simulink model "VIRTUAL_self_driving_stack_autoLocalize_v2"  (R2026a)
settings: Solver=ode1  StopTime=inf  FixedStep=1/500  EnableMultiTasking=on
values from neighbouring files (symbols this model uses):
  path_x4 = [-0.614 -0.604 -0.594 -0.584 -0.574 -0.564 -0.554 -0.544 -0.534 -0.524 -0.514 -0.504 ... (1761 elements, 1761x1)]    [SDCS_Paths_7.mat]
  path_y4 = [-1.0887 -1.0887 -1.0887 -1.0887 -1.0887 -1.0887 -1.0887 -1.0887 -1.0887 -1.0887 -1.0887 -1.0887 ... (1761 elements, 1761x1)]    [SDCS_Paths_7.mat]
undefined symbols (not defined in the file or in its folder): AAAF5050, CSI_Sample_Time, DiscIntNeverNeededParam, gcbh, height, HIL, ImageDisplay_Sample_Time, Initialization_Time, JPEG, K12, left, LiDAR_Sample_Time, MC, qc_get_step_size, RealSense_Sample_Time, top, video_display_show, width
libraries: quarc_library x67, simulink x5, visionconversions x1, visiontransforms x1, sl_discontinuities x1
(part 2 of 3)

== system VIRTUAL_self_driving_stack_autoLocalize_v2/readQCarDAC ==
  HIL Initialize : quarc_library/Data Acquisition/Generic/Configuration/HIL Initialize  object_name=HIL-2  board_type=qcar2  board_number=0@tcpip://localhost:18960  board_options=gyro_fs=250;gyro_rate=500;gyro_bw=125;gyro_ord=3;accel_fs=4;accel_rate=500;accel_bw=250;accel_ord=3;temp_bw=4000;enc0_dir=0;enc1_dir=0;enc2_dir=0;steer_bias=0.05;  exclusive=off  active=on  hardware_clocks=[]  clock_modes=[]  initial_clock_frequencies=[]  set_clock_params_at_start=off  set_clock_params_at_switch_in=off  set_clock_frequencies_at_start=off  set_clock_frequencies_at_switch_in=off  analog_input_channels=[0:4]  analog_input_configurations=[]  analog_input_maximums=[3.3]  analog_input_minimums=[0]  set_analog_input_params_at_start=off  set_analog_input_params_at_switch_in=off  analog_output_channels=[]  analog_output_maximums=[]  analog_output_minimums=[]  initial_analog_outputs=[]  final_analog_outputs=[]  watchdog_analog_outputs=[]  set_analog_output_params_at_start=off  set_analog_output_params_at_switch_in=off  set_analog_outputs_at_start=off  set_analog_outputs_at_switch_in=off  set_analog_outputs_at_terminate=off  set_analog_outputs_at_switch_out=off  set_analog_outputs_on_watchdog=off  digital_input_channels=[0:14]  digital_output_channels=[11:26]  digital_output_configuration=[]  initial_digital_outputs=[0]  final_digital_outputs=[0]  watchdog_digital_outputs=[0]  set_digital_output_params_at_start=off  set_digital_output_params_at_switch_in=off  set_digital_outputs_at_start=on  set_digital_outputs_at_switch_in=off  set_digital_outputs_at_terminate=on  set_digital_outputs_at_switch_out=off  set_digital_outputs_on_watchdog=off  encoder_channels=[0:2]  quadrature=[4]  encoder_filter_frequency=100e6/1  initial_encoder_counts=[0]  set_encoder_params_at_start=on  set_encoder_params_at_switch_in=off  set_encoder_counts_at_start=on  set_encoder_counts_at_switch_in=off  pwm_channels=[0:1]  pwm_modes=[0]  pwm_frequency=180e6/4096  pwm_configuration=[0]  pwm_alignment=[0]  pwm_polarity=[1]  pwm_leading_deadband=[]  pwm_trailing_deadband=[]  initial_pwm_outputs=[0]  final_pwm_outputs=[0]  watchdog_pwm_outputs=[0]  set_pwm_params_at_start=on  set_pwm_params_at_switch_in=off  set_pwm_outputs_at_start=on  set_pwm_outputs_at_switch_in=off  set_pwm_outputs_at_terminate=on  set_pwm_outputs_at_switch_out=off  set_pwm_outputs_on_watchdog=off  other_output_channels=[1000 11000]  initial_other_outputs=[0]  final_other_outputs=[0]  watchdog_other_outputs=[0]  set_other_outputs_at_start=on  set_other_outputs_at_switch_in=off  set_other_outputs_at_terminate=on  set_other_outputs_at_switch_out=off  set_other_outputs_on_watchdog=off
  HIL Read Timebase : quarc_library/Data Acquisition/Generic/Timebases/HIL Read Timebase  object_name=HIL-2  clock=0  analog_channels=[4 2]  encoder_channels=[0]  digital_channels=[]  other_channels=[3000:3002 4000:4002 14000]  active=on  vector_output=off  port_labels=channel numbers  data_type_mode=Inherit via back propagation  encoder_data_type=double  digital_data_type=boolean  overflow_mode=Synchronize (for simulated cards only)  samples_in_buffer=max(ceil(1/qc_get_step_size), 1)
  Mux1 : Mux  Inputs=3
  Mux2 : Mux  Inputs=3
  Unwrap 2^24 : quarc_library/Discontinuities/Inverse Modulus  modulus=16777215  output_derivative=off  output_revolutions=off  max_x=Inf  min_x=-Inf
  counts to meters : Subsystem
  counts/s to m/s : Subsystem
  powerConsumptionMonitor : Subsystem
  Speed (m/s) : Outport  VectorParamsAs1DForOutWhenUnconnected=off
  accelerometer (m/s^2) : Outport  Port=2  VectorParamsAs1DForOutWhenUnconnected=off
  gyroscope (rad/s) : Outport  Port=3  VectorParamsAs1DForOutWhenUnconnected=off
  odometer (m) : Outport  Port=4  VectorParamsAs1DForOutWhenUnconnected=off
  batteryVoltage (V) : Outport  Port=5
  motorCurrent (A) : Outport  Port=6
  batteryLevel (%) : Outport  Port=7
  motorPower (W) : Outport  Port=8
  wires:
  HIL Read Timebase/3 -> Unwrap 2^24/1  "encoder counts"
  HIL Read Timebase/1 -> powerConsumptionMonitor/1(motorCurrent (A) [1]), motorCurrent (A)/1  "motor current"
  HIL Read Timebase/2 -> batteryVoltage (V)/1, powerConsumptionMonitor/2(batteryVoltage (V) [1])  "battery voltage"
  HIL Read Timebase/10 -> counts/s to m/s/1(motorSpeed (counts/s))
  Unwrap 2^24/1 -> counts to meters/1(motorSpeed (counts/s))
  counts to meters/1(longitudinalCarSpeed (m/s)) -> odometer (m)/1
  counts/s to m/s/1(longitudinalCarSpeed (m/s)) -> Speed (m/s)/1
  powerConsumptionMonitor/1(motorPowerConsumption (W) [1]) -> motorPower (W)/1
  powerConsumptionMonitor/2(batteryLevel (%) [1]) -> batteryLevel (%)/1
  HIL Read Timebase/4 -> Mux1/1  "x"
  HIL Read Timebase/5 -> Mux1/2  "y"
  HIL Read Timebase/6 -> Mux1/3  "z"
  Mux1/1 -> gyroscope (rad/s)/1
  HIL Read Timebase/7 -> Mux2/1  "x"
  HIL Read Timebase/8 -> Mux2/2  "y"
  HIL Read Timebase/9 -> Mux2/3  "z"
  Mux2/1 -> accelerometer (m/s^2)/1

== system VIRTUAL_self_driving_stack_autoLocalize_v2/realsenseCapture ==
  Terminator{,1..4} (5 alike) : Terminator
  Video3D Initialize : quarc_library/Multimedia/Video3D Initialize  object_name=RealSense  source=Device  identifier=0@tcpip://localhost:18965  file=sample.bag  sample_time=RealSense_Sample_Time  active=on
  realsenseDepthCapture : quarc_library/Multimedia/Video3D Capture  object_name=RealSense  stream_type=Depth  stream_index=0  resolution=640 x 480  width=640  height=480  output_format=Distance in meters (HxW)  data_type=single  sample_time=RealSense_Sample_Time  camera_intrinsics=off  depth_scale=off  brightness_override=Do not override  brightness=50.0  contrast_override=Do not override  contrast=50.0  hue_override=Do not override  hue=50.0  saturation_override=Do not override  saturation=50.0  sharpness_override=Do not override  sharpness=50.0  gamma_override=Do not override  gamma=50.0  gain_override=Do not override  gain=50.0  backlightcompensation_override=Do not override  backlightcompensation=50.0  whitebalance_override=Automatic white balance  whitebalance=50.0  exposure_override=Automatic exposure  exposure=30.0  emitter=Enable laser emitter  preset=Do not set camera presets
  realsenseRGBCapture : quarc_library/Multimedia/Video3D Capture  object_name=RealSense  stream_type=RGB  stream_index=0  resolution=640 x 480  width=640  height=480  output_format=MATLAB RGB (HxWx3)  data_type=uint8  sample_time=RealSense_Sample_Time*1  camera_intrinsics=off  depth_scale=off  brightness_override=Do not override  brightness=50.0  contrast_override=Do not override  contrast=50.0  hue_override=Do not override  hue=50.0  saturation_override=Do not override  saturation=50.0  sharpness_override=Do not override  sharpness=50.0  gamma_override=Do not override  gamma=50.0  gain_override=Do not override  gain=50.0  backlightcompensation_override=Do not override  backlightcompensation=50.0  whitebalance_override=Automatic white balance  whitebalance=50.0  exposure_override=Automatic exposure  exposure=30.0  emitter=Enable laser emitter  preset=Do not set camera presets
  realsenseDepthImage [480 x 640] (single) : Outport
  newDepthImage [1] (bool) : Outport  Port=2
  "realsenseRGBImage [480 x 640] (uint8) " : Outport  Port=3
  newRGBImage [1] (bool) : Outport  Port=4
  wires:
  realsenseDepthCapture/4 -> newDepthImage [1] (bool)/1
  realsenseDepthCapture/2 -> Terminator4/1
  realsenseDepthCapture/3 -> Terminator3/1
  Video3D Initialize/1 -> Terminator/1
  realsenseRGBCapture/2 -> Terminator1/1
  realsenseRGBCapture/3 -> Terminator2/1
  realsenseRGBCapture/4 -> newRGBImage [1] (bool)/1
  realsenseRGBCapture/1 -> "realsenseRGBImage [480 x 640] (uint8) "/1
  realsenseDepthCapture/1 -> realsenseDepthImage [480 x 640] (single)/1

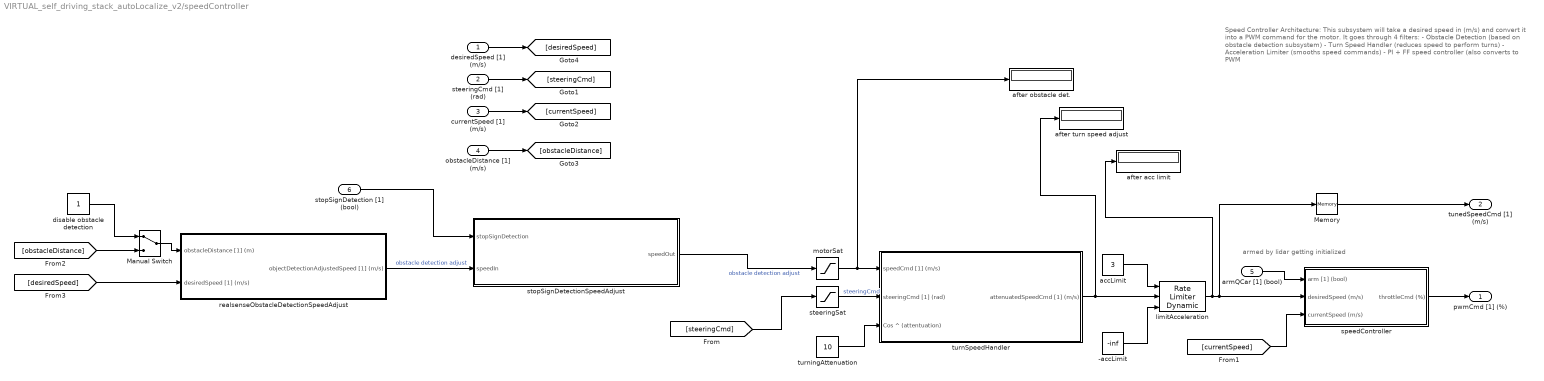
== system VIRTUAL_self_driving_stack_autoLocalize_v2/speedController ==
  note: Speed Controller Architecture:
      |
      | This subsystem will take a desired speed in (m/s) and convert it into a PWM command for the motor.
      |
      | It goes through 4 filters:
      | - Obstacle Detection (based on obstacle detection subsystem)
      | - Turn Speed Handler (reduces speed to perform turns)
      | - Acceleration Limiter (smooths speed commands)
      | - PI + FF speed controller (also converts to PWM
  note: armed by lidar getting initialized
  desiredSpeed [1] (m/s) : Inport
  steeringCmd [1] (rad) : Inport  Port=2
  currentSpeed [1] (m/s) : Inport  Port=3
  obstacleDistance [1] (m/s) : Inport  Port=4
  armQCar [1] (bool) : Inport  Port=5
  stopSignDetection [1] (bool) : Inport  Port=6
  -accLimit : Constant  Value=-inf
  Manual Switch : ManualSwitch
  Memory : Memory
  accLimit : Constant  Value=3
  after acc limit : Display
  after obstacle det. : Display
  after turn speed adjust : Display
  disable obstacle detection : Constant
  limitAcceleration : sl_discontinuities/Rate Limiter Dynamic
  motorSat : Saturate  UpperLimit=3  LowerLimit=-3
  realsenseObstacleDetectionSpeedAdjust : Subsystem
  speedController : Subsystem
  steeringSat : Saturate  UpperLimit=0.6  LowerLimit=-0.6
  stopSignDetectionSpeedAdjust : Subsystem
  turnSpeedHandler : Subsystem
  turningAttenuation : Constant  Value=10
  pwmCmd [1] (%) : Outport
  tunedSpeedCmd [1] (m/s) : Outport  Port=2
  wires:
  steeringSat/1 -> turnSpeedHandler/2(steeringCmd [1] (rad))  "steeringCmd"
  speedController/1(throttleCmd (%)) -> pwmCmd [1] (%)/1
  armQCar [1] (bool)/1 -> speedController/1(arm [1] (bool))
  turningAttenuation/1 -> turnSpeedHandler/3(Cos ^ (attentuation))
  motorSat/1 -> after obstacle det./1, turnSpeedHandler/1(speedCmd [1] (m/s))
  turnSpeedHandler/1(attenuatedSpeedCmd [1] (m/s)) -> after turn speed adjust/1, limitAcceleration/2
  accLimit/1 -> limitAcceleration/1
  limitAcceleration/1 -> after acc limit/1, Memory/1, speedController/2(desiredSpeed (m/s))
  -accLimit/1 -> limitAcceleration/3
  Memory/1 -> tunedSpeedCmd [1] (m/s)/1
  steeringCmd [1] (rad)/1 -> [steeringCmd]
  currentSpeed [1] (m/s)/1 -> [currentSpeed]
  [steeringCmd] -> steeringSat/1
  obstacleDistance [1] (m/s)/1 -> [obstacleDistance]
  [currentSpeed] -> speedController/3(currentSpeed (m/s))
  desiredSpeed [1] (m/s)/1 -> [desiredSpeed]
  [desiredSpeed] -> realsenseObstacleDetectionSpeedAdjust/2(desiredSpeed [1] (m/s))
  [obstacleDistance] -> Manual Switch/2
  disable obstacle detection/1 -> Manual Switch/1
  Manual Switch/1 -> realsenseObstacleDetectionSpeedAdjust/1(obstacleDistance [1] (m))
  stopSignDetection [1] (bool)/1 -> stopSignDetectionSpeedAdjust/1(stopSignDetection)
  realsenseObstacleDetectionSpeedAdjust/1(objectDetectionAdjustedSpeed [1] (m/s)) -> stopSignDetectionSpeedAdjust/2(speedIn)  "obstacle detection adjust"
  stopSignDetectionSpeedAdjust/1(speedOut) -> motorSat/1  "obstacle detection adjust"

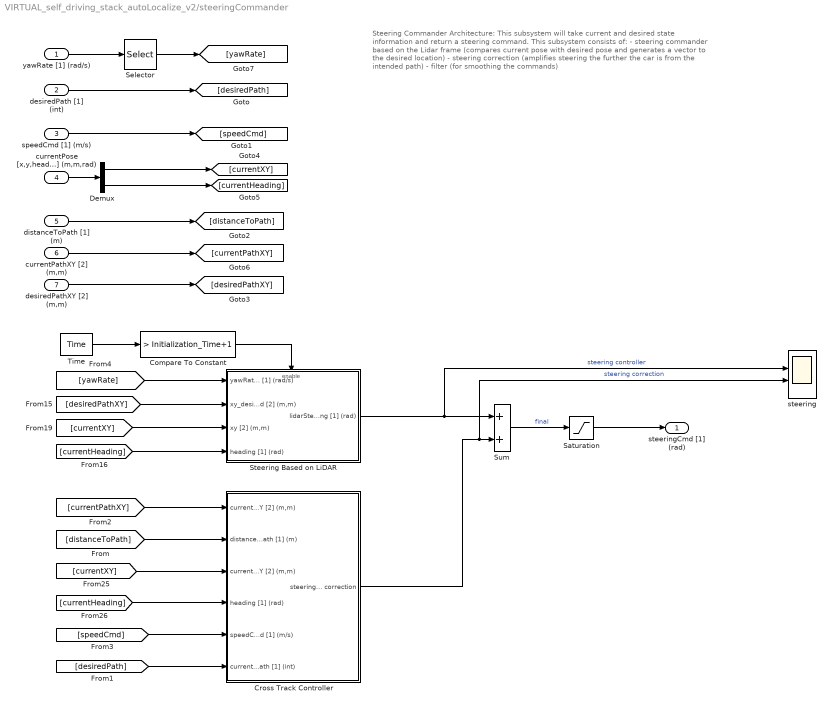
== system VIRTUAL_self_driving_stack_autoLocalize_v2/steeringCommander ==
  note: Steering Commander Architecture:
      |
      | This subsystem will take current and desired state information and return a steering command.
      |
      | This subsystem consists of:
      |
      | - steering commander based on the Lidar frame (compares current pose with desired pose and generates a vector to the desired location)
      | - steering correction (amplifies steering the further the car is from the intended path)
      | - filter (for smoothing the commands)
  yawRate [1] (rad/s) : Inport
  desiredPath [1] (int) : Inport  Port=2
  speedCmd [1] (m/s) : Inport  Port=3
  currentPose [x,y,heading] (m,m,rad) : Inport  Port=4
  distanceToPath [1] (m) : Inport  Port=5
  currentPathXY [2] (m,m) : Inport  Port=6
  desiredPathXY [2] (m,m) : Inport  Port=7
  Compare To Constant : simulink/Logic and Bit Operations/Compare To Constant  relop=>  const=Initialization_Time+1  OutDataTypeStr=boolean
  Cross Track Controller : Subsystem
  Demux : Demux  Outputs=2
  Saturation : Saturate
  Selector : Selector  InputPortWidth=3  IndexOptions=Index vector (dialog)  Indices=[3]  OutputSizes=1
  Steering Based on LiDAR : Subsystem
  Sum : Sum
  Time : quarc_library/Sources/Time/Time  time_source=Wall clock  sample_time=qc_get_step_size
  steering : Scope  NumInputPorts=4
      settings: ActiveDisplayYMinimum=-3.4883  ActiveDisplayYMaximum=3.496
  steeringCmd [1] (rad) : Outport
  wires:
  Demux/1 -> [currentXY]
  currentPose [x,y,heading] (m,m,rad)/1 -> Demux/1
  [desiredPathXY] -> Steering Based on LiDAR/2(xy_desired [2] (m,m))
  Steering Based on LiDAR/1(lidarSteering [1] (rad)) -> steering/2, Sum/1  "steering controller"
  [currentHeading] -> Cross Track Controller/4(heading [1] (rad))
  Demux/2 -> [currentHeading]
  [currentXY] -> Cross Track Controller/3(currentXY [2] (m,m))
  [currentXY] -> Steering Based on LiDAR/3(xy [2] (m,m))
  desiredPath [1] (int)/1 -> [desiredPath]
  [desiredPath] -> Cross Track Controller/6(currentPath [1] (int))
  speedCmd [1] (m/s)/1 -> [speedCmd]
  [speedCmd] -> Cross Track Controller/5(speedCmd [1] (m/s))
  Time/1 -> Compare To Constant/1
  Compare To Constant/1 -> Steering Based on LiDAR/Enable
  distanceToPath [1] (m)/1 -> [distanceToPath]
  desiredPathXY [2] (m,m)/1 -> [desiredPathXY]
  currentPathXY [2] (m,m)/1 -> [currentPathXY]
  [distanceToPath] -> Cross Track Controller/2(distanceToPath [1] (m))
  [currentPathXY] -> Cross Track Controller/1(currentPathXY [2] (m,m))
  Cross Track Controller/1(steering correction) -> steering/3, Sum/2  "steering correction"
  [currentHeading] -> Steering Based on LiDAR/4(heading [1] (rad))
  yawRate [1] (rad/s)/1 -> Selector/1
  [yawRate] -> Steering Based on LiDAR/1(yawRate [1] (rad/s))
  Selector/1 -> [yawRate]
  Sum/1 -> Saturation/1  "final"
  Saturation/1 -> steeringCmd [1] (rad)/1

== system VIRTUAL_self_driving_stack_autoLocalize_v2/writeToQCarDAC ==
  note: 11: LED left outside brake light
      | 12: LED left inside brake light
      | 12: LED right inside brake light
      | 13: LED right outside brake fight
      | 14: LED left reverse light
      | 15: LED right reverse light
      | 16: LED left rear signal
      | 17: LED right rear signal
      | 18: LED left outside headlight
      | 19: LED left middle headlight
      | 20: LED left inside headlight
      | 21: LED right inside headlight
      | 22: LED right middle headlight
      | 23: LED right outside headlight
      | 24: LED left front signal
      | 25: LED right front signal
  motor_cmd [1] (%) : Inport
  steering_cmd [1] (rad) : Inport  Port=2
  leds [14] (bool) : Inport  Port=3
  ledStrip [R,G,B] (%) : Inport  Port=4
  Gain : Gain
  HIL Write : quarc_library/Data Acquisition/Generic/Immediate I//O/HIL Write  object_name=HIL-2  analog_channels=[]  pwm_channels=[]  digital_channels=[11:26]  other_channels=[1000 11000]  sample_time=-1  active=on  vector_input=on  port_labels=channel numbers
  LED Strip1 : quarc_library/Devices/Third-Party/Displays/LED Strip  Commented=on  led_type=AAAF5050-MC-K12  uri=tcpip://localhost:18969  mode=individual  max_leds=33  initial_red=[0]  initial_green=[0]  initial_blue=[0]  final_red=[0]  final_green=[0]  final_blue=[0]  sample_time=-1  use_vectors=off  active=off
      settings: SourceProductName=QUARC Targets
  Mux : Mux  Inputs=2
  Steering Bias : Bias  Bias=-0.05  SaturateOnIntegerOverflow=off
  Terminator : Terminator
  motor sat : Saturate  UpperLimit=.6  LowerLimit=-0.6
  steering sat : Saturate
  wires:
  ledStrip [R,G,B] (%)/1 -> LED Strip1/1
  steering_cmd [1] (rad)/1 -> Steering Bias/1
  motor sat/1 -> Mux/2
  steering sat/1 -> Mux/1
  leds [14] (bool)/1 -> HIL Write/1
  Steering Bias/1 -> Gain/1
  motor_cmd [1] (%)/1 -> motor sat/1
  LED Strip1/1 -> Terminator/1
  Gain/1 -> steering sat/1
  Mux/1 -> HIL Write/2

== system VIRTUAL_self_driving_stack_autoLocalize_v2/CSICameras/Video Compressed Display ==
  In1 : Inport
  Channel : quarc_library/Signal Routing/Channel  channel=0  buffer_size=1
  Image Compress : quarc_library/Image Processing/Generic/Image Compress  algorithm=JPEG  source=Internal dialog parameter  quality=quality  output_dim=-1
  Video Display : quarc_library/Multimedia/Video Display  Tag=quarc_library/Multimedia/Video Compressed Display/Video Display  sample_time=sample_time  use_hardware=on
  wires:
  Image Compress/1 -> Channel/1
  In1/1 -> Image Compress/1
  Channel/1 -> Video Display/1

== system VIRTUAL_self_driving_stack_autoLocalize_v2/CSICameras/Video Compressed Display1 ==
  In1 : Inport
  Channel : quarc_library/Signal Routing/Channel  channel=1  buffer_size=1
  Image Compress : quarc_library/Image Processing/Generic/Image Compress  algorithm=JPEG  source=Internal dialog parameter  quality=quality  output_dim=-1
  Video Display : quarc_library/Multimedia/Video Display  Tag=quarc_library/Multimedia/Video Compressed Display/Video Display  sample_time=sample_time  use_hardware=on
  wires:
  Channel/1 -> Video Display/1
  In1/1 -> Image Compress/1
  Image Compress/1 -> Channel/1

== system VIRTUAL_self_driving_stack_autoLocalize_v2/CSICameras/Video Compressed Display2 ==
  In1 : Inport
  Channel : quarc_library/Signal Routing/Channel  channel=2  buffer_size=1
  Image Compress : quarc_library/Image Processing/Generic/Image Compress  algorithm=JPEG  source=Internal dialog parameter  quality=quality  output_dim=-1
  Video Display : quarc_library/Multimedia/Video Display  Tag=quarc_library/Multimedia/Video Compressed Display/Video Display  sample_time=sample_time  use_hardware=on
  wires:
  Image Compress/1 -> Channel/1
  In1/1 -> Image Compress/1
  Channel/1 -> Video Display/1

== system VIRTUAL_self_driving_stack_autoLocalize_v2/CSICameras/Video Compressed Display3 ==
  In1 : Inport
  Channel : quarc_library/Signal Routing/Channel  channel=3  buffer_size=1
  Image Compress : quarc_library/Image Processing/Generic/Image Compress  algorithm=JPEG  source=Internal dialog parameter  quality=quality  output_dim=-1
  Video Display : quarc_library/Multimedia/Video Display  Tag=quarc_library/Multimedia/Video Compressed Display/Video Display  sample_time=sample_time  use_hardware=on
  wires:
  Channel/1 -> Video Display/1
  In1/1 -> Image Compress/1
  Image Compress/1 -> Channel/1

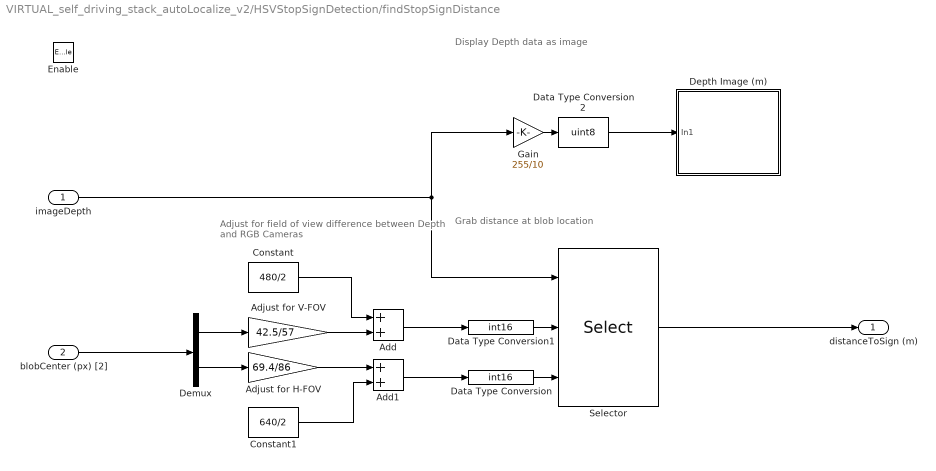
== system VIRTUAL_self_driving_stack_autoLocalize_v2/HSVStopSignDetection/findStopSignDistance ==
  note: Grab distance at blob location
  note: Display Depth data as image
  note: Adjust for field of view difference
      | between Depth and RGB Cameras
  imageDepth : Inport
  blobCenter (px) [2] : Inport  Port=2
  Enable : EnablePort  PropagateVarSize=During execution
  Add : Sum
  Add1 : Sum
  Adjust for H-FOV : Gain  Gain=69.4/86
  Adjust for V-FOV : Gain  Gain=42.5/57
  Constant : Constant  Value=480/2
  Constant1 : Constant  Value=640/2
  Data Type Conversion : DataTypeConversion  OutDataTypeStr=int16  SaturateOnIntegerOverflow=off  RndMeth=Floor
  Data Type Conversion1 : DataTypeConversion  OutDataTypeStr=int16  SaturateOnIntegerOverflow=off  RndMeth=Floor
  Data Type Conversion2 : DataTypeConversion  OutDataTypeStr=uint8  SaturateOnIntegerOverflow=off  RndMeth=Floor
  Demux : Demux  Outputs=2
  Depth Image (m) : Subsystem  LoadFcn=set_param(gcbh, 'UserData', gcb);  StartFcn=video_display_show([gcb, '/Video Display'], 'add', gcb);  mask(Video Compressed Display){algorithm=JPEG, quality=50, sample_time=-1, use_hardware=on}
      mask prompts: algorithm "Compression algorithm:"; quality "Compression quality (0-100):"; sample_time "Sample time (seconds):"; use_hardware "Use hardware acceleration for video display"
      mask help: Displays a video stream on the host, using compression to minimize bandwidth.
      mask init:
      | qc_set_display('Video\nCompressed\nDisplay');
      settings: UndoDeleteFcn=set_param(gcbh, 'UserData', gcb);  OpenFcn=video_display_show([gcb, '/Video Display'], 'show', gcb);  PreDeleteFcn=video_display_show([gcb, '/Video Display'], 'delete');
      settings: CopyFcn=|
      | set_param(gcbh, 'UserData', gcb);
      | set_param(gcbh, 'LinkStatus', 'none');
      settings: NameChangeFcn=|
      | video_display_show([get_param(gcbh, 'UserData'), '/Video Display'], 'rename', [gcb, '/Video Display']);
      | video_display_show([gcb, '/Video Display'], 'add', gcb);
      | set_param(gcbh, 'UserData', gcb);
      mask Help: web(qc_get_block_help_path(gcb));
      mask TypeOptions algorithm: Image Compress/algorithm
      mask TypeOptions quality: Image Compress/quality
      mask TypeOptions sample_time: Video Display/sample_time
      mask TypeOptions use_hardware: Video Display/use_hardware
      mask Display:
      | patch([0.98591 0.98591 0.62618 0.59072 0.56147   0.536   0.536  0.5441 0.56912 0.59207 0.60881 0.62276 0.63527 0.64364  0.6485  0.6485 0.64706 0.64499 0.63662 0.62411 0.61232 0.59837 0.58307 0.56147   0.536   0.536  0.5441  0.5747 0.60953 0.63662 0.67001  0.7034 0.72851 0.75425 0.77927 0.80294 0.82454 0.84119 0.85865 0.87395 0.88574 0.89339  0.8969 0.89969 0.89969 0.89267  0.8816 0.87044 0.85649  0.8384 0.81824 0.80294 0.78764 0.77513 0.76676 0.75776 0.76397 0.77513 0.79178 0.80987 0.82796 0.84326 0.86207 0.98528],[0.18689 0.05522 0.05522 0.05171 0.05171    0.05 0.18338 0.18338 0.19148 0.20435 0.22298 0.24863 0.28589 0.33125 0.38138 0.55139 0.59801 0.63761 0.68189 0.72149 0.74939 0.76694 0.77855 0.79367 0.79952 0.92768 0.92768 0.92768 0.92417 0.92066 0.91364  0.9032 0.89384 0.88106 0.86594 0.85073 0.82634 0.80537 0.77855 0.74363 0.70403 0.65858 0.61079 0.59099 0.41513 0.37202 0.31847 0.29048 0.25556 0.23342  0.2102 0.19382 0.18221 0.17285 0.16943 0.16124  0.1589 0.16241 0.16709 0.17168  0.1787 0.18221 0.18689 0.18689],[0.9,0.90,0.91])
      | patch([0.536 0.52601 0.46823 0.44528 0.41603 0.39101 0.35555 0.33116 0.31451 0.29291  0.2804 0.26717 0.25322 0.23999 0.22406 0.20732 0.19337 0.17528 0.15935 0.14396 0.13217 0.11759 0.10922 0.10085 0.09671 0.09392 0.09041 0.08906 0.08906 0.09464  0.0995 0.10778 0.11894 0.13145 0.14675 0.16349 0.17672 0.19409 0.20732 0.22406 0.23999 0.26159 0.27833 0.29849 0.31793 0.33602 0.35411 0.37085 0.39245 0.41603   0.536   0.536 0.53159 0.46409   0.446 0.42026 0.39587 0.37571 0.36113 0.34925 0.34088 0.33809 0.33809 0.34088 0.34583 0.35627 0.36392 0.38129 0.39587 0.41117 0.42719 0.44672  0.4676 0.48353 0.48353 0.52394   0.536],[0.05 0.04829 0.04712 0.04712 0.04829 0.05063 0.05405 0.05873 0.06107 0.06692 0.07043 0.07619 0.08087 0.08672 0.09482 0.10652 0.11696 0.13325  0.1508 0.17168 0.19499 0.22415 0.25439 0.28472 0.31379 0.35456 0.38489 0.41513 0.58055 0.63878 0.68774 0.72149 0.75641 0.78089 0.80537 0.82859 0.84029 0.85658 0.86594 0.87404  0.8834 0.89267 0.90086 0.90788 0.91247 0.91832 0.92066   0.923 0.92651 0.92768 0.92768 0.79952 0.79952 0.79952 0.79718 0.78899 0.77153 0.75056 0.72149 0.68072 0.62249  0.5549 0.41396 0.37085 0.33242 0.28121 0.25205 0.22181 0.20552 0.19499 0.18572 0.18221 0.17753 0.17636 0.17753  0.1787  0.1787],[0.9,0.90,0.91])
      | disp('Video\nCompressed\nDisplay');
  Gain : Gain  Gain=255/10
  Selector : Selector  NumberOfDimensions=2  InputPortWidth=3  IndexOptions=Index vector (port),Index vector (port)  Indices=[1 3],1  OutputSizes=1,1
  distanceToSign (m) : Outport  VectorParamsAs1DForOutWhenUnconnected=off
  wires:
  blobCenter (px) [2]/1 -> Demux/1
  Demux/2 -> Adjust for H-FOV/1
  Adjust for V-FOV/1 -> Add/2
  Adjust for H-FOV/1 -> Add1/1
  Data Type Conversion/1 -> Selector/3
  Data Type Conversion1/1 -> Selector/2
  Add/1 -> Data Type Conversion1/1
  Constant/1 -> Add/1
  Constant1/1 -> Add1/2
  Demux/1 -> Adjust for V-FOV/1
  Add1/1 -> Data Type Conversion/1
  Gain/1 -> Data Type Conversion2/1
  imageDepth/1 -> Gain/1, Selector/1
  Data Type Conversion2/1 -> Depth Image (m)/1(In1)
  Selector/1 -> distanceToSign (m)/1

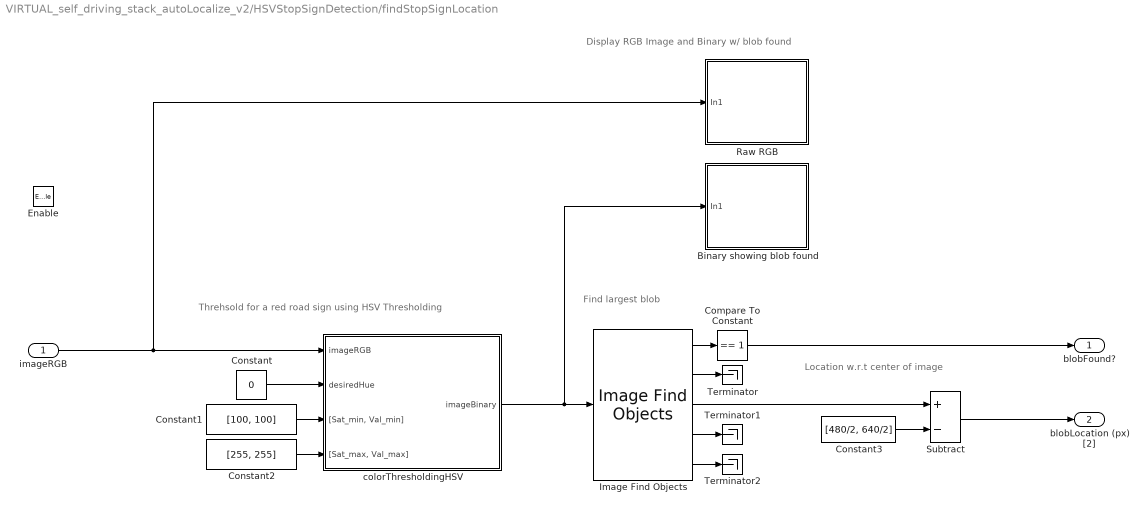
== system VIRTUAL_self_driving_stack_autoLocalize_v2/HSVStopSignDetection/findStopSignLocation ==
  note: Location w.r.t center of image
  note: Find largest blob
  note: Threhsold for a red road sign using HSV Thresholding
  note: Display RGB Image and Binary w/ blob found
  imageRGB : Inport
  Enable : EnablePort  PropagateVarSize=During execution
  Binary showing blob found : Subsystem  LoadFcn=set_param(gcbh, 'UserData', gcb);  StartFcn=video_display_show([gcb, '/Video Display'], 'add', gcb);  mask(Video Compressed Display){algorithm=JPEG, quality=50, sample_time=-1, use_hardware=on}
      mask prompts: algorithm "Compression algorithm:"; quality "Compression quality (0-100):"; sample_time "Sample time (seconds):"; use_hardware "Use hardware acceleration for video display"
      mask help: Displays a video stream on the host, using compression to minimize bandwidth.
      mask init:
      | qc_set_display('Video\nCompressed\nDisplay');
      settings: UndoDeleteFcn=set_param(gcbh, 'UserData', gcb);  OpenFcn=video_display_show([gcb, '/Video Display'], 'show', gcb);  PreDeleteFcn=video_display_show([gcb, '/Video Display'], 'delete');
      settings: CopyFcn=|
      | set_param(gcbh, 'UserData', gcb);
      | set_param(gcbh, 'LinkStatus', 'none');
      settings: NameChangeFcn=|
      | video_display_show([get_param(gcbh, 'UserData'), '/Video Display'], 'rename', [gcb, '/Video Display']);
      | video_display_show([gcb, '/Video Display'], 'add', gcb);
      | set_param(gcbh, 'UserData', gcb);
      mask Help: web(qc_get_block_help_path(gcb));
      mask TypeOptions algorithm: Image Compress/algorithm
      mask TypeOptions quality: Image Compress/quality
      mask TypeOptions sample_time: Video Display/sample_time
      mask TypeOptions use_hardware: Video Display/use_hardware
      mask Display:
      | patch([0.98591 0.98591 0.62618 0.59072 0.56147   0.536   0.536  0.5441 0.56912 0.59207 0.60881 0.62276 0.63527 0.64364  0.6485  0.6485 0.64706 0.64499 0.63662 0.62411 0.61232 0.59837 0.58307 0.56147   0.536   0.536  0.5441  0.5747 0.60953 0.63662 0.67001  0.7034 0.72851 0.75425 0.77927 0.80294 0.82454 0.84119 0.85865 0.87395 0.88574 0.89339  0.8969 0.89969 0.89969 0.89267  0.8816 0.87044 0.85649  0.8384 0.81824 0.80294 0.78764 0.77513 0.76676 0.75776 0.76397 0.77513 0.79178 0.80987 0.82796 0.84326 0.86207 0.98528],[0.18689 0.05522 0.05522 0.05171 0.05171    0.05 0.18338 0.18338 0.19148 0.20435 0.22298 0.24863 0.28589 0.33125 0.38138 0.55139 0.59801 0.63761 0.68189 0.72149 0.74939 0.76694 0.77855 0.79367 0.79952 0.92768 0.92768 0.92768 0.92417 0.92066 0.91364  0.9032 0.89384 0.88106 0.86594 0.85073 0.82634 0.80537 0.77855 0.74363 0.70403 0.65858 0.61079 0.59099 0.41513 0.37202 0.31847 0.29048 0.25556 0.23342  0.2102 0.19382 0.18221 0.17285 0.16943 0.16124  0.1589 0.16241 0.16709 0.17168  0.1787 0.18221 0.18689 0.18689],[0.9,0.90,0.91])
      | patch([0.536 0.52601 0.46823 0.44528 0.41603 0.39101 0.35555 0.33116 0.31451 0.29291  0.2804 0.26717 0.25322 0.23999 0.22406 0.20732 0.19337 0.17528 0.15935 0.14396 0.13217 0.11759 0.10922 0.10085 0.09671 0.09392 0.09041 0.08906 0.08906 0.09464  0.0995 0.10778 0.11894 0.13145 0.14675 0.16349 0.17672 0.19409 0.20732 0.22406 0.23999 0.26159 0.27833 0.29849 0.31793 0.33602 0.35411 0.37085 0.39245 0.41603   0.536   0.536 0.53159 0.46409   0.446 0.42026 0.39587 0.37571 0.36113 0.34925 0.34088 0.33809 0.33809 0.34088 0.34583 0.35627 0.36392 0.38129 0.39587 0.41117 0.42719 0.44672  0.4676 0.48353 0.48353 0.52394   0.536],[0.05 0.04829 0.04712 0.04712 0.04829 0.05063 0.05405 0.05873 0.06107 0.06692 0.07043 0.07619 0.08087 0.08672 0.09482 0.10652 0.11696 0.13325  0.1508 0.17168 0.19499 0.22415 0.25439 0.28472 0.31379 0.35456 0.38489 0.41513 0.58055 0.63878 0.68774 0.72149 0.75641 0.78089 0.80537 0.82859 0.84029 0.85658 0.86594 0.87404  0.8834 0.89267 0.90086 0.90788 0.91247 0.91832 0.92066   0.923 0.92651 0.92768 0.92768 0.79952 0.79952 0.79952 0.79718 0.78899 0.77153 0.75056 0.72149 0.68072 0.62249  0.5549 0.41396 0.37085 0.33242 0.28121 0.25205 0.22181 0.20552 0.19499 0.18572 0.18221 0.17753 0.17636 0.17753  0.1787  0.1787],[0.9,0.90,0.91])
      | disp('Video\nCompressed\nDisplay');
  Compare To Constant : simulink/Logic and Bit Operations/Compare To Constant  relop===  const=1  OutDataTypeStr=boolean
  Constant : Constant  Value=0
  Constant1 : Constant  Value=[100, 100]
  Constant2 : Constant  Value=[255, 255]
  Constant3 : Constant  Value=[480/2, 640/2]
  Image Find Objects : quarc_library/Image Processing/Generic/Image Find Objects  num_objects=1  connectivity=8 directions (N, NE, E, SE, S, SW, W, NW)  sort_order=Sort by bounding box area  min_pixels=100  max_pixels=intmax('uint32')  largest=on  exclude_at_edges=on  variable_size=off  use_complex=off
      settings: SourceProductName=QUARC Targets
  Raw RGB : Subsystem  LoadFcn=set_param(gcbh, 'UserData', gcb);  StartFcn=video_display_show([gcb, '/Video Display'], 'add', gcb);  mask(Video Compressed Display){algorithm=JPEG, quality=50, sample_time=-1, use_hardware=on}
      mask prompts: algorithm "Compression algorithm:"; quality "Compression quality (0-100):"; sample_time "Sample time (seconds):"; use_hardware "Use hardware acceleration for video display"
      mask help: Displays a video stream on the host, using compression to minimize bandwidth.
      mask init:
      | qc_set_display('Video\nCompressed\nDisplay');
      settings: UndoDeleteFcn=set_param(gcbh, 'UserData', gcb);  OpenFcn=video_display_show([gcb, '/Video Display'], 'show', gcb);  PreDeleteFcn=video_display_show([gcb, '/Video Display'], 'delete');
      settings: CopyFcn=|
      | set_param(gcbh, 'UserData', gcb);
      | set_param(gcbh, 'LinkStatus', 'none');
      settings: NameChangeFcn=|
      | video_display_show([get_param(gcbh, 'UserData'), '/Video Display'], 'rename', [gcb, '/Video Display']);
      | video_display_show([gcb, '/Video Display'], 'add', gcb);
      | set_param(gcbh, 'UserData', gcb);
      mask Help: web(qc_get_block_help_path(gcb));
      mask TypeOptions algorithm: Image Compress/algorithm
      mask TypeOptions quality: Image Compress/quality
      mask TypeOptions sample_time: Video Display/sample_time
      mask TypeOptions use_hardware: Video Display/use_hardware
      mask Display:
      | patch([0.98591 0.98591 0.62618 0.59072 0.56147   0.536   0.536  0.5441 0.56912 0.59207 0.60881 0.62276 0.63527 0.64364  0.6485  0.6485 0.64706 0.64499 0.63662 0.62411 0.61232 0.59837 0.58307 0.56147   0.536   0.536  0.5441  0.5747 0.60953 0.63662 0.67001  0.7034 0.72851 0.75425 0.77927 0.80294 0.82454 0.84119 0.85865 0.87395 0.88574 0.89339  0.8969 0.89969 0.89969 0.89267  0.8816 0.87044 0.85649  0.8384 0.81824 0.80294 0.78764 0.77513 0.76676 0.75776 0.76397 0.77513 0.79178 0.80987 0.82796 0.84326 0.86207 0.98528],[0.18689 0.05522 0.05522 0.05171 0.05171    0.05 0.18338 0.18338 0.19148 0.20435 0.22298 0.24863 0.28589 0.33125 0.38138 0.55139 0.59801 0.63761 0.68189 0.72149 0.74939 0.76694 0.77855 0.79367 0.79952 0.92768 0.92768 0.92768 0.92417 0.92066 0.91364  0.9032 0.89384 0.88106 0.86594 0.85073 0.82634 0.80537 0.77855 0.74363 0.70403 0.65858 0.61079 0.59099 0.41513 0.37202 0.31847 0.29048 0.25556 0.23342  0.2102 0.19382 0.18221 0.17285 0.16943 0.16124  0.1589 0.16241 0.16709 0.17168  0.1787 0.18221 0.18689 0.18689],[0.9,0.90,0.91])
      | patch([0.536 0.52601 0.46823 0.44528 0.41603 0.39101 0.35555 0.33116 0.31451 0.29291  0.2804 0.26717 0.25322 0.23999 0.22406 0.20732 0.19337 0.17528 0.15935 0.14396 0.13217 0.11759 0.10922 0.10085 0.09671 0.09392 0.09041 0.08906 0.08906 0.09464  0.0995 0.10778 0.11894 0.13145 0.14675 0.16349 0.17672 0.19409 0.20732 0.22406 0.23999 0.26159 0.27833 0.29849 0.31793 0.33602 0.35411 0.37085 0.39245 0.41603   0.536   0.536 0.53159 0.46409   0.446 0.42026 0.39587 0.37571 0.36113 0.34925 0.34088 0.33809 0.33809 0.34088 0.34583 0.35627 0.36392 0.38129 0.39587 0.41117 0.42719 0.44672  0.4676 0.48353 0.48353 0.52394   0.536],[0.05 0.04829 0.04712 0.04712 0.04829 0.05063 0.05405 0.05873 0.06107 0.06692 0.07043 0.07619 0.08087 0.08672 0.09482 0.10652 0.11696 0.13325  0.1508 0.17168 0.19499 0.22415 0.25439 0.28472 0.31379 0.35456 0.38489 0.41513 0.58055 0.63878 0.68774 0.72149 0.75641 0.78089 0.80537 0.82859 0.84029 0.85658 0.86594 0.87404  0.8834 0.89267 0.90086 0.90788 0.91247 0.91832 0.92066   0.923 0.92651 0.92768 0.92768 0.79952 0.79952 0.79952 0.79718 0.78899 0.77153 0.75056 0.72149 0.68072 0.62249  0.5549 0.41396 0.37085 0.33242 0.28121 0.25205 0.22181 0.20552 0.19499 0.18572 0.18221 0.17753 0.17636 0.17753  0.1787  0.1787],[0.9,0.90,0.91])
      | disp('Video\nCompressed\nDisplay');
  Subtract : Sum  Inputs=+-
  Terminator : Terminator
  Terminator1 : Terminator
  Terminator2 : Terminator
  colorThresholdingHSV : Subsystem
  blobFound? : Outport  VectorParamsAs1DForOutWhenUnconnected=off
  blobLocation (px) [2] : Outport  Port=2  VectorParamsAs1DForOutWhenUnconnected=off
  wires:
  Constant/1 -> colorThresholdingHSV/2(desiredHue)
  Constant1/1 -> colorThresholdingHSV/3("[Sat_min, Val_min]")
  Constant2/1 -> colorThresholdingHSV/4("[Sat_max, Val_max]")
  colorThresholdingHSV/1(imageBinary) -> Binary showing blob found/1(In1), Image Find Objects/1
  Image Find Objects/1 -> Compare To Constant/1
  Image Find Objects/2 -> Terminator/1
  Image Find Objects/4 -> Terminator1/1
  Image Find Objects/5 -> Terminator2/1
  imageRGB/1 -> Raw RGB/1(In1), colorThresholdingHSV/1(imageRGB)
  Compare To Constant/1 -> blobFound?/1
  Image Find Objects/3 -> Subtract/1
  Subtract/1 -> blobLocation (px) [2]/1
  Constant3/1 -> Subtract/2

== system VIRTUAL_self_driving_stack_autoLocalize_v2/YOLOStopSignDetection/Edge Detection ==
  realsenseRGBImage : Inport
  Image Filter : quarc_library/Image Processing/Generic/Image Filter  filter_type=Sobel  source_of_roi=Internal dialog parameter  roi_style=[top, left, height, width]  roi=[]  maximum_roi=[]  roi_zone=Operate inside region of interest  border_type=Replicate  border_value=[0 0 0]  kernel_size=5  sigma=10  mask_size=[3 3]  kernel=int16([-2 -1 0; -1 1 1; 0 1 2])  divisor=1  offset=0  rounding=Nearest  algorithm_hint=None  threshold=100  alpha=0.9  num_frames=8  num_valid=1  gap_threshold=10  depth_threshold=255  iterations=2  norm_type=L1
      settings: AttributesFormatString=(%<filter_type>)  SourceProductName=QUARC Targets
  Out1 : Outport
  wires:
  Image Filter/1 -> Out1/1
  realsenseRGBImage/1 -> Image Filter/1

== system VIRTUAL_self_driving_stack_autoLocalize_v2/YOLOStopSignDetection/Hough Transform ==
  realsenseRGBImage : Inport
  Autothreshold : visionconversions/Autothreshold  operator=>  threshOut=off  effMetricOut=off  userDefinedRange=off  umin=0  umax=255  outOfRngOpt=Ignore  scaleThreshold=off  scaleFactor=1  roundingMode=Floor  overflowMode=off  P1Mode=Specify word length  P1WordLength=32  P1FracLength=30  P2Mode=Specify word length  P2WordLength=32  P2FracLength=22  P3Mode=Specify word length  P3WordLength=32  P3FracLength=14  P4Mode=Binary point scaling  P4WordLength=32  P4FracLength=15  Q1Mode=Specify word length  Q1WordLength=32  Q1FracLength=16  EMMode=Specify word length  EMWordLength=16  EMFracLength=14
  Hough Transform : visiontransforms/Hough Transform  theta_res=pi/180  rho_res=1  out_theta_rho=on  outdtmode=double  roundingMode=Nearest  overflowMode=on  firstCoeffMode=Binary point scaling  firstCoeffWordLength=16  firstCoeffFracLength=14  secondCoeffMode=Binary point scaling  secondCoeffWordLength=32  secondCoeffFracLength=16  prodOutputMode=Binary point scaling  prodOutputWordLength=32  prodOutputFracLength=20  accumMode=Binary point scaling  accumWordLength=32  accumFracLength=20  outputMode=Binary point scaling  outputWordLength=16  outputFracLength=0  memoryMode=Binary point scaling  memoryWordLength=32  memoryFracLength=16
  Image Convert : quarc_library/Image Processing/Generic/Image Convert  input_format=MATLAB RGB (HxWx3)  padding=0  output_format=MATLAB greyscale (HxW)  data_type=uint8
      settings: AttributesFormatString=(%<input_format>)  SourceProductName=QUARC Targets
  Terminator5 : Terminator
  Terminator6 : Terminator
  Terminator7 : Terminator
  Out1 : Outport
  wires:
  Hough Transform/2 -> Terminator6/1
  Autothreshold/1 -> Out1/1, Hough Transform/1
  Hough Transform/3 -> Terminator7/1
  Image Convert/1 -> Autothreshold/1
  Hough Transform/1 -> Terminator5/1
  realsenseRGBImage/1 -> Image Convert/1

== system VIRTUAL_self_driving_stack_autoLocalize_v2/YOLOStopSignDetection/Subsystem ==
  realsenseDepthImage : Inport
  realsenseRGBImage : Inport  Port=2
  Distance in Meters : MATLABSystem  System=RoadYOLODistance  SimulateUsing=Interpreted execution
      mask Type: RoadYOLODistance
  YOLO v4 Detector : MATLABSystem  System=RoadYOLODetector  ModelFile=road_yolo_detector.mat  Threshold=0.35  MaxDetections=100  ExecutionEnvironment=cpu  SimulateUsing=Interpreted execution
      mask Type: RoadYOLODetector
  distances : Outport
  confidence scores : Outport  Port=2
  lane coordinates : Outport  Port=3
  annot output : Outport  Port=4
  wires:
  Distance in Meters/1 -> distances/1
  YOLO v4 Detector/5 -> Distance in Meters/4
  YOLO v4 Detector/4 -> Distance in Meters/3
  YOLO v4 Detector/2 -> Distance in Meters/2
  realsenseRGBImage/1 -> YOLO v4 Detector/1
  YOLO v4 Detector/1 -> annot output/1
  realsenseDepthImage/1 -> Distance in Meters/1
  YOLO v4 Detector/6 -> lane coordinates/1
  YOLO v4 Detector/3 -> confidence scores/1

== system VIRTUAL_self_driving_stack_autoLocalize_v2/localization/Subsystem ==
  Angle : Inport
  Bias : Bias  Bias=pi  SaturateOnIntegerOverflow=off
  Bias1 : Bias  Bias=-pi  SaturateOnIntegerOverflow=off
  Constant1 : Constant  Value=2*pi
  Mod : Math  Operator=mod
  Mod_Angle : Outport
  wires:
  Angle/1 -> Bias/1
  Bias1/1 -> Mod_Angle/1
  Bias/1 -> Mod/1
  Constant1/1 -> Mod/2
  Mod/1 -> Bias1/1

== system VIRTUAL_self_driving_stack_autoLocalize_v2/obstacleDetection/Newer Depth ==
  In1 : Inport
  Channel : quarc_library/Signal Routing/Channel  channel=0  buffer_size=1
  Image Compress : quarc_library/Image Processing/Generic/Image Compress  algorithm=JPEG  source=Internal dialog parameter  quality=quality  output_dim=-1
  Video Display : quarc_library/Multimedia/Video Display  Tag=VIRTUAL_self_driving_stack_autoLocalize/obstacleDetection/Newer Depth/Video Display  sample_time=sample_time  use_hardware=on
  wires:
  Image Compress/1 -> Channel/1
  In1/1 -> Image Compress/1
  Channel/1 -> Video Display/1

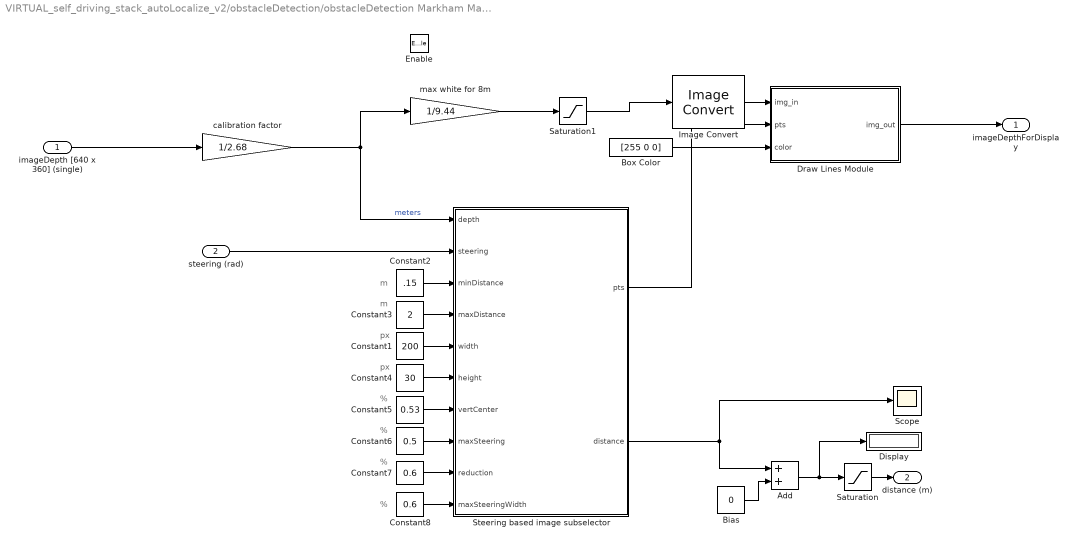
== system VIRTUAL_self_driving_stack_autoLocalize_v2/obstacleDetection/obstacleDetection Markham March 22 ==
  note: %
  note: m
  note: m
  note: %
  note: px
  note: px
  note: %
  note: %
  imageDepth [640 x 360] (single) : Inport
  steering (rad) : Inport  Port=2
  Enable : EnablePort  PropagateVarSize=During execution
  Add : Sum
  Bias : Constant  Value=0
  Box Color : Constant  Value=[255 0 0]
  Constant1 : Constant  Value=200
  Constant2 : Constant  Value=.15
  Constant3 : Constant  Value=2
  Constant4 : Constant  Value=30
  Constant5 : Constant  Value=0.53
  Constant6 : Constant  Value=0.5
  Constant7 : Constant  Value=0.6
  Constant8 : Constant  Value=0.6
  Display : Display
  Draw Lines Module : MATLAB Function  TreatAsAtomicUnit=on
  Image Convert : quarc_library/Image Processing/Generic/Image Convert  input_format=MATLAB greyscale (HxW)  padding=0  output_format=MATLAB greyscale (HxW)  data_type=uint16
      settings: AttributesFormatString=(%<input_format>)  SourceProductName=QUARC Targets
  Saturation : Saturate  UpperLimit=2  LowerLimit=0.05
  Saturation1 : Saturate  UpperLimit=1  LowerLimit=0
  Scope : Scope
  Steering based image subselector : MATLAB Function  TreatAsAtomicUnit=on
  calibration factor : Gain  Gain=1/2.68
  max white for 8m : Gain  Gain=1/9.44
  imageDepthForDisplay : Outport  VectorParamsAs1DForOutWhenUnconnected=off
  distance (m) : Outport  Port=2  VectorParamsAs1DForOutWhenUnconnected=off
  wires:
  Saturation1/1 -> Image Convert/1
  Constant6/1 -> Steering based image subselector/8(maxSteering)
  Steering based image subselector/2(distance) -> Add/1, Scope/1
  Constant5/1 -> Steering based image subselector/7(vertCenter)
  Constant4/1 -> Steering based image subselector/6(height)
  Constant1/1 -> Steering based image subselector/5(width)
  Constant3/1 -> Steering based image subselector/4(maxDistance)
  Constant2/1 -> Steering based image subselector/3(minDistance)
  steering (rad)/1 -> Steering based image subselector/2(steering)
  Draw Lines Module/1(img_out) -> imageDepthForDisplay/1
  Steering based image subselector/1(pts) -> Draw Lines Module/2(pts)
  Image Convert/1 -> Draw Lines Module/1(img_in)
  max white for 8m/1 -> Saturation1/1
  imageDepth [640 x 360] (single)/1 -> calibration factor/1
  Bias/1 -> Add/2
  Add/1 -> Saturation/1, Display/1
  Saturation/1 -> distance (m)/1
  Box Color/1 -> Draw Lines Module/3(color)
  Constant7/1 -> Steering based image subselector/9(reduction)
  Constant8/1 -> Steering based image subselector/10(maxSteeringWidth)
  calibration factor/1 -> Steering based image subselector/1(depth), max white for 8m/1  "meters"

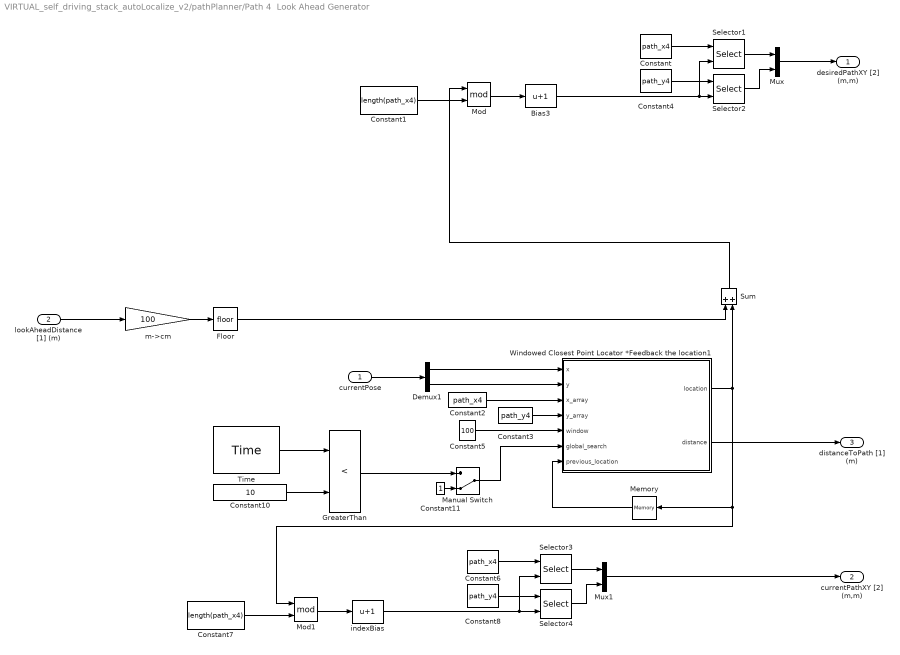
== system VIRTUAL_self_driving_stack_autoLocalize_v2/pathPlanner/Path 4  Look Ahead Generator ==
  currentPose : Inport
  lookAheadDistance [1] (m) : Inport  Port=2
  Bias3 : Bias  Bias=1  SaturateOnIntegerOverflow=off
  Constant : Constant  Value=path_x4
  Constant1 : Constant  Value=length(path_x4)
  Constant10 : Constant  Value=10
  Constant11 : Constant
  Constant2 : Constant  Value=path_x4
  Constant3 : Constant  Value=path_y4
  Constant4 : Constant  Value=path_y4
  Constant5 : Constant  Value=100
  Constant6 : Constant  Value=path_x4
  Constant7 : Constant  Value=length(path_x4)
  Constant8 : Constant  Value=path_y4
  Demux1 : Demux  Outputs=2
  Floor : Rounding
  GreaterThan : RelationalOperator  Operator=<  OutDataTypeStr=boolean  RndMeth=Simplest  InputSameDT=off
  Manual Switch : ManualSwitch  CurrentSetting=0
  Memory : Memory  InitialCondition=1  InheritSampleTime=on  LinearizeMemory=on  LinearizeAsDelay=on
  Mod : Math  Operator=mod
  Mod1 : Math  Operator=mod
  Mux : Mux  Inputs=2
  Mux1 : Mux  Inputs=2
  Selector{1..4} (4 alike) : Selector  InputPortWidth=length(path_x4)  IndexOptions=Index vector (port)  Indices=[1 3]  OutputSizes=1
  Sum : Sum
  Time : quarc_library/Sources/Time/Time  time_source=Wall clock  sample_time=qc_get_step_size
  Windowed Closest Point Locator *Feedback the location1 : MATLAB Function  TreatAsAtomicUnit=on
  indexBias : Bias  Bias=1  SaturateOnIntegerOverflow=off
  m->cm : Gain  Gain=100
  desiredPathXY [2] (m,m) : Outport
  currentPathXY [2] (m,m) : Outport  Port=2
  distanceToPath [1] (m) : Outport  Port=3
  wires:
  Windowed Closest Point Locator *Feedback the location1/1(location) -> Mod1/1, Memory/1, Sum/2
  Memory/1 -> Windowed Closest Point Locator *Feedback the location1/7(previous_location)
  Constant5/1 -> Windowed Closest Point Locator *Feedback the location1/5(window)
  Bias3/1 -> Selector2/2, Selector1/2
  Windowed Closest Point Locator *Feedback the location1/2(distance) -> distanceToPath [1] (m)/1
  Selector2/1 -> Mux/2
  Mux/1 -> desiredPathXY [2] (m,m)/1
  Constant4/1 -> Selector2/1
  Selector1/1 -> Mux/1
  Constant/1 -> Selector1/1
  Floor/1 -> Sum/1
  m->cm/1 -> Floor/1
  lookAheadDistance [1] (m)/1 -> m->cm/1
  currentPose/1 -> Demux1/1
  Mod/1 -> Bias3/1
  Demux1/2 -> Windowed Closest Point Locator *Feedback the location1/2(y)
  Sum/1 -> Mod/1
  Constant1/1 -> Mod/2
  Constant3/1 -> Windowed Closest Point Locator *Feedback the location1/4(y_array)
  Constant2/1 -> Windowed Closest Point Locator *Feedback the location1/3(x_array)
  Demux1/1 -> Windowed Closest Point Locator *Feedback the location1/1(x)
  Mux1/1 -> currentPathXY [2] (m,m)/1
  Mod1/1 -> indexBias/1
  Selector4/1 -> Mux1/2
  Constant7/1 -> Mod1/2
  Selector3/1 -> Mux1/1
  Constant8/1 -> Selector4/1
  indexBias/1 -> Selector3/2, Selector4/2
  Constant6/1 -> Selector3/1
  Time/1 -> GreaterThan/1
  Constant10/1 -> GreaterThan/2
  Manual Switch/1 -> Windowed Closest Point Locator *Feedback the location1/6(global_search)
  Constant11/1 -> Manual Switch/2
  GreaterThan/1 -> Manual Switch/1

== system VIRTUAL_self_driving_stack_autoLocalize_v2/pathPlanner/rateAligner ==
  xy 1 : Inport
  xy 2 : Inport  Port=2
  Demux1 : Demux  Outputs=2
  Demux2 : Demux  Outputs=2
  Mux : Mux  Inputs=2
  Mux1 : Mux  Inputs=2
  Rate Transition1 : RateTransition  OutPortSampleTime=ImageDisplay_Sample_Time
  Rate Transition2 : RateTransition  OutPortSampleTime=ImageDisplay_Sample_Time
  x : Outport
  y : Outport  Port=2
  wires:
  Demux2/1 -> Mux/2
  Demux1/2 -> Mux1/1
  Demux1/1 -> Mux/1
  Demux2/2 -> Mux1/2
  Mux/1 -> x/1
  Mux1/1 -> y/1
  xy 1/1 -> Rate Transition1/1
  Rate Transition1/1 -> Demux1/1
  xy 2/1 -> Rate Transition2/1
  Rate Transition2/1 -> Demux2/1

== system VIRTUAL_self_driving_stack_autoLocalize_v2/rateTimingPlots/monitorTiming ==
  note: Timing Performance
  note: moniorTiming Module:
      |
      | This subsystem outputs the sample time and computation time of the model.
      |
      | Outputs:
      | sampleTime (s) n/a : Sample time (unfiltered and filtered) in seconds.
      | computationTime (s) n/a : Computation time (unfiltered and filtered) in seconds.
      |
      | Usage:
      | Compare the Sample Time (s) output to a constant (qc_get_step_size) to monitor whether or not the desired sample time is being achieved. The Computation Time (s) values should be lower than the corresponding sample time value to ensure that the solver has enough time per time step.
  Computation Time : quarc_library/Sources/Time/Computation Time  sample_time=CSI_Sample_Time  use_model=on  use_cpu_time=off
  Constant : Constant  Value=CSI_Sample_Time  SampleTime=-1
  Mux : Mux  Inputs=3
  Sample Time : quarc_library/Sources/Time/Sample Time  Priority=-99  sample_time=CSI_Sample_Time
  Timing (s) : Outport  VectorParamsAs1DForOutWhenUnconnected=off
  wires:
  Computation Time/1 -> Mux/3
  Mux/1 -> Timing (s)/1
  Sample Time/1 -> Mux/1
  Constant/1 -> Mux/2

== system VIRTUAL_self_driving_stack_autoLocalize_v2/rateTimingPlots/monitorTiming1 ==
  note: moniorTiming Module:
      |
      | This subsystem outputs the sample time and computation time of the model.
      |
      | Outputs:
      | sampleTime (s) n/a : Sample time (unfiltered and filtered) in seconds.
      | computationTime (s) n/a : Computation time (unfiltered and filtered) in seconds.
      |
      | Usage:
      | Compare the Sample Time (s) output to a constant (qc_get_step_size) to monitor whether or not the desired sample time is being achieved. The Computation Time (s) values should be lower than the corresponding sample time value to ensure that the solver has enough time per time step.
  note: Timing Performance
  Computation Time : quarc_library/Sources/Time/Computation Time  sample_time=qc_get_step_size  use_model=on  use_cpu_time=off
  Constant : Constant  Value=qc_get_step_size  SampleTime=-1
  Mux : Mux  Inputs=3
  Sample Time : quarc_library/Sources/Time/Sample Time  Priority=-99  sample_time=qc_get_step_size
  Timing (s) : Outport  VectorParamsAs1DForOutWhenUnconnected=off
  wires:
  Constant/1 -> Mux/2
  Sample Time/1 -> Mux/1
  Mux/1 -> Timing (s)/1
  Computation Time/1 -> Mux/3

== system VIRTUAL_self_driving_stack_autoLocalize_v2/rateTimingPlots/monitorTiming2 ==
  note: moniorTiming Module:
      |
      | This subsystem outputs the sample time and computation time of the model.
      |
      | Outputs:
      | sampleTime (s) n/a : Sample time (unfiltered and filtered) in seconds.
      | computationTime (s) n/a : Computation time (unfiltered and filtered) in seconds.
      |
      | Usage:
      | Compare the Sample Time (s) output to a constant (qc_get_step_size) to monitor whether or not the desired sample time is being achieved. The Computation Time (s) values should be lower than the corresponding sample time value to ensure that the solver has enough time per time step.
  note: Timing Performance
  Computation Time : quarc_library/Sources/Time/Computation Time  sample_time=RealSense_Sample_Time  use_model=on  use_cpu_time=off
  Constant : Constant  Value=RealSense_Sample_Time  SampleTime=-1
  Mux : Mux  Inputs=3
  Sample Time : quarc_library/Sources/Time/Sample Time  Priority=-99  sample_time=RealSense_Sample_Time
  Timing (s) : Outport  VectorParamsAs1DForOutWhenUnconnected=off
  wires:
  Constant/1 -> Mux/2
  Sample Time/1 -> Mux/1
  Mux/1 -> Timing (s)/1
  Computation Time/1 -> Mux/3

== system VIRTUAL_self_driving_stack_autoLocalize_v2/rateTimingPlots/monitorTiming3 ==
  note: Timing Performance
  note: moniorTiming Module:
      |
      | This subsystem outputs the sample time and computation time of the model.
      |
      | Outputs:
      | sampleTime (s) n/a : Sample time (unfiltered and filtered) in seconds.
      | computationTime (s) n/a : Computation time (unfiltered and filtered) in seconds.
      |
      | Usage:
      | Compare the Sample Time (s) output to a constant (qc_get_step_size) to monitor whether or not the desired sample time is being achieved. The Computation Time (s) values should be lower than the corresponding sample time value to ensure that the solver has enough time per time step.
  Computation Time : quarc_library/Sources/Time/Computation Time  sample_time=ImageDisplay_Sample_Time  use_model=on  use_cpu_time=off
  Constant : Constant  Value=ImageDisplay_Sample_Time  SampleTime=-1
  Mux : Mux  Inputs=3
  Sample Time : quarc_library/Sources/Time/Sample Time  Priority=-99  sample_time=ImageDisplay_Sample_Time
  Timing (s) : Outport  VectorParamsAs1DForOutWhenUnconnected=off
  wires:
  Computation Time/1 -> Mux/3
  Mux/1 -> Timing (s)/1
  Sample Time/1 -> Mux/1
  Constant/1 -> Mux/2
